simulink model "oc4_VarMass"  (R2026a)
settings: Solver=ode4  StartTime=0  StopTime=400  FixedStep=0.1  MaxStep=0.1  EnableMultiTasking=on
values from neighbouring files (symbols this model uses):
  simu = simulationClass()    [wecSimInputFile.m]
  waves = waveClass('regular')    [wecSimInputFile.m]
undefined symbols (not defined in the file or in its folder): body, constraint, X, Y, Z
libraries: nesl_utility x22, sm_lib x12, WECSim_Lib_Body_Elements x4, vrlib x1, matrix_library x1, WECSim_Lib_Constraints x1, WECSim_Lib_Frames x1
(part 1 of 3)
settings Model: Creator=mlawson  LastModifiedBy=jniffene
settings SolverCC: ZeroCrossControl=DisableAll  AlgebraicLoopSolver=LineSearch
settings OptimizationCC: SimCompilerOptimization=on
settings HardwareCC: ProdHWDeviceType=32-bit Generic
settings SimscapeCC: SimscapeNormalizeSystem=off  SimscapeNominalValues="[{\"value\":\"1\",\"unit\":\"A\"},{\"value\":\"1\",\"unit\":\"bar\"},{\"value\":\"1\",\"unit\":\"cm^2\"},{\"value\":\"1\",\"unit\":\"cm^3/s\"},{\"value\":\"1\",\"unit\":\"kJ/kg\"},{\"value\":\"1\",\"unit\":\"kW\"},{\"value\":\"1\",\"unit\":\"l\"},{\"value\":\"1\",\"unit\":\"N\"},{\"value\":\"1\",\"unit\":\"N*m\"},{\"value\":\"1\",\"unit\":\"V\"}]"  SimscapeLogType=none  SimscapeLogDataHistory=5000.0
settings ConfigurationSet: Description=SimMechanics 2G
settings ExplorerConfigSet: InternalSimMechanicsExplorerSettings="<ExplorerConfiguration><canonicalview>default</canonicalview><TilePanel><TileInfo><Tiles Columns=\"1\" Count=\"1\" Rows=\"1\"><Column Left=\"2\" Weight=\"1\"/><Column Left=\"1335\"/><Row Top=\"2\" Weight=\"1\"/><Row Top=\"911\"/><Tile Height=\"1\" Width=\"1\" X=\"0\" Y=\"0\"/></Tiles></TileInfo><SceneInfo><SceneViewer><BGColor><R>0.60000002384185791</R><G>0.60000002384185791</G><B>0.60000002384185791</B></BGColor><Camera><Position><X>365.37645888990272</X><Y>-369.82486814446582</Y><Z>359.64809521743916</Z></Position><Center><X>-6.7351450971904585</X><Y>2.2867358426280204</Y><Z>-12.463508769654169</Z></Center><Up><X>-0.40824829046386307</X><Y>0.40824829046386307</Y><Z>0.81649658092772615</Z></Up><Left>-57.820127362122818</Left><Right>57.820127362122818</Right><Bottom>-38.308817187253304</Bottom><Top>38.308817187253304</Top></Camera></SceneViewer></SceneInfo></TilePanel></ExplorerConfiguration>"

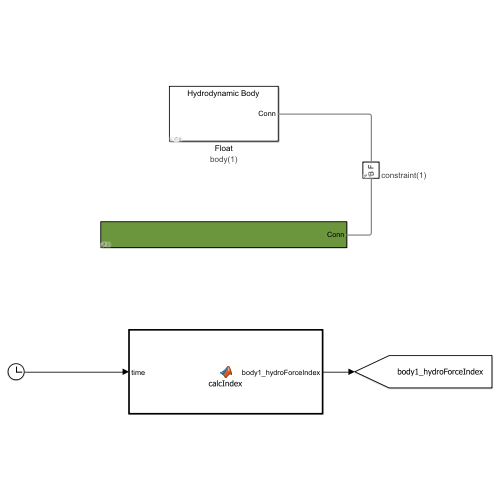
[thumbnail: Simulink's stored preview of the top-level diagram]
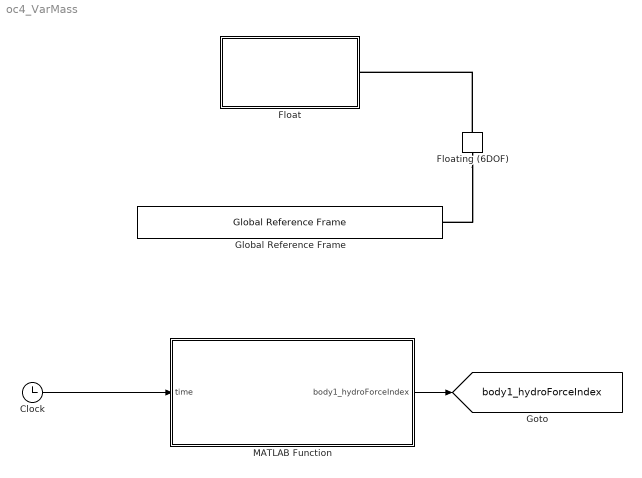
== system oc4_VarMass ==
  Clock : Clock
  Float : Subsystem  AncestorBlock=WECSim_Lib_Body_Elements/Rigid Body  Variant=on  EmptyChoice=on  mask(Rigid Body){body=body(1)}
      mask prompts: body "Body Number:"
      mask help:
      | A rigid body has no generalized body modes. It can be a standard hydrodynamic body, a drag body, or a non-hydrodynamic body.
      |
      | The variable name input below must be 'body(i)' where i=1,2,...
      | body(i) must be defined in the input file with the fields appropriate to each variant.
      mask init:
      | if exist('body','var')
      |     %%
      |     % Hydro Body
      |     h = [gcb '/Hydrodynamic Body'];
      |     responseName = ['sv_b' num2str(body.number) '_hydroBody'];
      |     set_param(h,'VariantControl',responseName);
      |     %%
      |     % Hydro Body Morison Element: Off
      |     h = [gcb '/Hydrodynamic Body/Morison Element and Viscous Damping Force Calculation/Morison Element Variant Subsystem/Morison Element Off'];
      |     responseName = ['sv_b' num2str(body.number) '_MEOff'];
      |     set_param(h,'VariantControl',responseName);
      |     %%
      |     % Hydro Body Morison Element: On
      |     h = [gcb '/Hydrodynamic Body/Morison Element and Viscous Damping Force Calculation/Morison Element Variant Subsystem/Morison Element On'];
      |     responseName = ['sv_b' num2str(body.number) '_MEOn'];
      |     set_param(h,'VariantControl',responseName);
      |     %%
      |     % Hydro Body Nonlinear Froude Krylov Force: Off
      |     h = [gcb '/Hydrodynamic Body/Wave Diffraction and Excitation Force Calculation/Nonlinear FK Force Variant Subsystem/No Nonlinear FroudeKrylov Force'];
      |     responseName = ['sv_b' num2str(body.number) '_linearHydro'];
      |     set_param(h,'VariantControl',responseName);
      |     %%
      |     % Hydro Body Nonlinear Froude Krylov Force: On
      |     h = [gcb '/Hydrodynamic Body/Wave Diffraction and Excitation Force Calculation/Nonlinear FK Force Variant Subsystem/With Nonlinear FroudeKrylov Force'];
      |     responseName = ['sv_b' num2str(body.number) '_nonlinearHydro'];
      |     set_param(h,'VariantControl',responseName);
      |     %%
      |     % Hydro Body Nonlinear Restoring: Off
      |     h = [gcb '/Hydrodynamic Body/Hydrostatic Restoring Force Calculation/Linear and Nonlinear Restoring Force Variant Subsystem/Linear Hydrostatic Restoring Force'];
      |     responseName = ['sv_b' num2str(body.number) '_linearHydro'];
      |     set_param(h,'VariantControl',responseName);
      |     %%
      |     % Hydro Body Nonlinear Restoring: On
      |     h = [gcb '/Hydrodynamic Body/Hydrostatic Restoring Force Calculation/Linear and Nonlinear Restoring Force Variant Subsystem/Nonlinear Hydrostatic Restoring Force'];
      |     responseName = ['sv_b' num2str(body.number) '_nonlinearHydro'];
      |     set_param(h,'VariantControl',responseName);
      |     %%
      |     % Hydro Body Regular Excitation Passive Yaw: Off
      |     h = [gcb '/Hydrodynamic Body/Wave Diffraction and Excitation Force Calculation/Linear Wave Excitation Force Variant Subsystem/Regular Wave ' newline 'Excitation Force'];
      |     responseName = ['sv_regularWaves_b' num2str(body.number)];
      |     set_param(h,'VariantControl',responseName);
      |     %%
      |     % Hydro Body Regular Excitation Passive Yaw: On
      |     h = [gcb '/Hydrodynamic Body/Wave Diffraction and Excitation Force Calculation/Linear Wave Excitation Force Variant Subsystem/Regular Wave ' newline 'NonLinear Yaw'];
      |     responseName = ['sv_regularWavesYaw_b' num2str(body.number)];
      |     set_param(h,'VariantControl',responseName);
      |     %%    
      |     % Hydro Body Irregular Excitation Passive Yaw: Off
      |     h = [gcb '/Hydrodynamic Body/Wave Diffraction and Excitation Force Calculation/Linear Wave Excitation Force Variant Subsystem/Irregular Wave ' newline 'Excitation Force'];
      |     responseName = ['sv_irregularWaves_b' num2str(body.number)];
      |     set_param(h,'VariantControl',responseName);
      |     %%
      |     % Hydro Body Irregular Excitation Passive Yaw: On
      |     h = [gcb '/Hydrodynamic Body/Wave Diffraction and Excitation Force Calculation/Linear Wave Excitation Force Variant Subsystem/Irregular Wave ' newline 'NonLinearYaw'];
      |     responseName = ['sv_irregularWavesYaw_b' num2str(body.number)];
      |     set_param(h,'VariantControl',responseName);
      |     %%
      |     % Hydro Body Nonlinear Froude Krylov or Restoring: Instantaneous Free Surface
      |     h = [gcb '/Hydrodynamic Body/Nonlinear Wave Elevation/Linear or Instantaneous Free Surface/Instantaneous Water Free Surface'];
      |     responseName = ['sv_b' num2str(body.number) '_instFS'];
      |     set_param(h,'VariantControl',responseName);
      |     %%
      |     % Hydro Body Nonlinear Froude Krylov or Restoring: Mean Free Surface
      |     h = [gcb '/Hydrodynamic Body/Nonlinear Wave Elevation/Linear or Instantaneous Free Surface/Mean Water Free Surface'];
      |     responseName = ['sv_b' num2str(body.number) '_meanFS'];
      |     set_param(h,'VariantControl',responseName);
      |     %% Variable hydro on/off
      |     % Variable hydro control - variable hydro off
      |     h = [gcb '/Hydrodynamic Body/Variable Hydrodynamics Control/Variable Hydrodynamics Subsystem/noVariableHydro'];
      |     responseName = ['sv_b' num2str(body.number) '_noVariableHydro'];
      |     set_param(h,'VariantControl',responseName);
      |     % Variable hydro control - variable hydro on
      |     h = [gcb '/Hydrodynamic Body/Variable Hydrodynamics Control/Variable Hydrodynamics Subsystem/variableHydro'];
      |     responseName = ['sv_b' num2str(body.number) '_variableHydro'];
      |     set_param(h,'VariantControl',responseName);
      |     % CIC - variable hydro off
      |     h = [gcb '/Hydrodynamic Body/Wave Radiation Forces Calculation/SS CI and Constant-Damping-CoeVariant Subsystem/Convolution Integral Calculation/Convolution Variant Subsystem/Convolution Integral Calculation'];
      |     responseName = ['sv_b' num2str(body.number) '_noVariableHydro'];
      |     set_param(h,'VariantControl',responseName);
      |     % CIC - variable hydro on
      |     h = [gcb '/Hydrodynamic Body/Wave Radiation Forces Calculation/SS CI and Constant-Damping-CoeVariant Subsystem/Convolution Integral Calculation/Convolution Variant Subsystem/Convolution Integral Surface Calculation'];
      |     responseName = ['sv_b' num2str(body.number) '_variableHydro'];
      |     set_param(h,'VariantControl',responseName);
      |     %%
      |     % Drag Body
      |     h = [gcb '/Drag Body'];
      |     responseName = ['sv_b' num2str(body.number) '_dragBody'];
      |     set_param(h,'VariantControl',responseName);
      |     %%
      |     % Drag Body Morison Element: Off
      |     h = [gcb '/Drag Body/Morison Element and Viscous Damping Force Calculation/Morison Element Variant Subsystem/Morison Element Off'];
      |     responseName = ['sv_b' num2str(body.number) '_MEOff'];
      |     set_param(h,'VariantControl',responseName);
      |     %%
      |     % Drag Body Morison Element: On
      |     h = [gcb '/Drag Body/Morison Element and Viscous Damping Force Calculation/Morison Element Variant Subsystem/Morison Element On'];
      |     responseName = ['sv_b' num2str(body.number) '_MEOn'];
      |     set_param(h,'VariantControl',responseName);
      |     %% 
      |     % Hydro Body QTF: Off
      |     h = [gcb '/Hydrodynamic Body/Wave Diffraction and Excitation Force Calculation/Second Order Excitation Force Variant Subsystem/No Second Order Excitation Force'];
      |     responseName = ['sv_b' num2str(body.number) '_noSecondOrderExt'];
      |     set_param(h,'VariantControl',responseName);
      |     %%
      |     % Hydro Body QTF: On
      |     h = [gcb '/Hydrodynamic Body/Wave Diffraction and Excitation Force Calculation/Second Order Excitation Force Variant Subsystem/With Second Order Excitation Force'];
      |     responseName = ['sv_b' num2str(body.number) '_secondOrderExt'];
      |     set_param(h,'VariantControl',responseName);
      |     %%
      |     % Set zero active variant controls to prevent label issue
      |     set_param(gcb,'AllowZeroVariantControls','on');
      | end
      | clear bc h geomFile responseName
      settings: AttributesFormatString=%<body>
      mask Help:
      | A rigid body has no generalized body modes. It can be a standard hydrodynamic body, a drag body, or a non-hydrodynamic body.
      | 
      | The variable name input below must be 'body(i)' where i=1,2,...
      | body(i) must be defined in the input file with the fields appropriate to each variant.
  Floating (6DOF) : WECSim_Lib_Constraints/Floating (6DOF)  constraint=constraint(1)
      settings: AttributesFormatString=%<constraint>
  Global Reference Frame : WECSim_Lib_Frames/Global Reference Frame  waves=waves  simu=simu
  MATLAB Function : MATLAB Function  TreatAsAtomicUnit=on
  tag scope: body1_hydroForceIndex=global
  wires:
  MATLAB Function/1(body1_hydroForceIndex) -> [body1_hydroForceIndex]
  Clock/1 -> MATLAB Function/1(time)
  connections:
  Floating (6DOF)/LConn1 -- Global Reference Frame/RConn1
  Floating (6DOF)/RConn1 -- Float/RConn1

== system oc4_VarMass/Float ==
  note: 1) Add Subsystem or Model blocks as valid variant choices.
      | 2) You cannot connect blocks at this level. At simulation, connectivity is automatically
      | determined, based on the active variant and port name matching.
  Drag Body : Subsystem  VariantControl=sv_b1_dragBody  mask(Drag Body){body=body}
      mask prompts: body "Body Name:"
      mask help:
      | A drag body contains six degrees of freedom in x, y, z and Mx, My, Mz. It contains a buoyant force, linear damping force, and Morison Element and viscous forces. It is not influenced by wave excitation, radiation damping or radiation added mass.
      |
      | The variable name input below must be 'body(i)' where i=1,2,...
      | body(i) must be defined in the input file with the following fields:
      |
      |     .mass (required)
      |             Float or string.
      |             The translational interia or mass of the body in kg. If a string, the value must be 'equilibrium'. Default = [ ]
      |     .momOfIntertia (required)
      |             3x1 vector [Ixx Iyy Izz].
      |             Rotational intertia of the body in kg*m^2. Default = [ ]
      |     .filename (required)
      |             String.
      |             The file path specifying the .h5 file for the body.
      |     .name (optional)
      |             String.
      |             Specifies the body name. Default = [ ]
      |     .cg (optional)
      |             3x1 float vector [x y z]
      |     .cb (optional)
      |             3x1 float vector [x y z]
      |             Body center of buoyancy in m. Default = [ ].
      |     .dispVol (optional)
      |             Float.
      |             Displaced volume at the equilibrium position in m^3. Default = [ ]
      |     .geometryFile (optional)
      |             String
      |             Path to the geometry file of the body (.stl). Required for nonlinear hydrodynamics or visualization. Default = [ ]
      mask init:
      | if exist('body','var')
      |     % geometry file name
      |     h=[gcb '/Structure/Body Properties'];
      |     geomFile=body.geometryFile;
      |     set_param(h,'ExtGeomFileName',geomFile);
      |     geomType='STL';
      |     % split version e.g. '9.10.0.16028 (R2021a)' into 9, 10, 0, NaN.
      |     % cannot compare str2double('9.10') because it becomes '9.1' 
      |     ver=split(version,'.');
      |     ver=str2double(ver(1:3));
      |     if ver(1) < 9 || (ver(1) == 9 && ver(2) < 6)
      |        set_param(h,'ExtGeomFileType',geomType);
      |     end
      |     % toWorkSpace: outputs
      |     h=[gcb '/To Workspace'];
      |     responseName=['body' num2str(body.number) '_out'];
      |     set_param(h,'VariableName',responseName);
      |     % position GoTo 
      |     h=[gcb '/Goto'];
      |     responseName=['disp' num2str(body.number)];
      |     set_param(h,'GotoTag',responseName);
      |     % position From
      |     h=[gcb '/From'];
      |     responseName=['disp' num2str(body.number)];
      |     set_param(h,'GotoTag',responseName);
      |     % velocity GoTo 
      |     h=[gcb '/Goto1'];
      |     responseName=['vel' num2str(body.number)];
      |     set_param(h,'GotoTag',responseName);
      |     % velocity From 
      |     h=[gcb '/From1'];
      |     responseName=['vel' num2str(body.number)];
      |     set_param(h,'GotoTag',responseName);
      |     % acceleration GoTo 
      |     h=[gcb '/Goto2'];
      |     responseName=['acc' num2str(body.number)];
      |     set_param(h,'GotoTag',responseName);
      |     % acceleration From 
      |     h=[gcb '/From2'];
      |     responseName=['acc' num2str(body.number)];
      |     set_param(h,'GotoTag',responseName);
      | end
  Hydrodynamic Body : Subsystem  VariantControl=sv_b1_hydroBody  mask(Hydrodynamic Body){body=body}
      mask prompts: body "Body Name:"
      mask help:
      | A Hydrodynamic Body contains six degrees of freedom in x, y, z and Mx, My, Mz. All wave forces interact with a hydrodynamic body.
      |
      | The variable name input below must be 'body(i)' where i=1,2,...
      | body(i) must be defined in the input file with the following fields:
      |
      |     .filename (required)
      |             String.
      |             The file path specifying the .h5 file for the body.
      |     .mass (required)
      |             Float or string.
      |             The translational interia or mass of the body in kg. If a string, the value must be 'equilibrium'. Default = [ ]
      |     .momOfIntertia (required)
      |             3x1 vector [Ixx Iyy Izz].
      |             Rotational intertia of the body in kg*m^2. Default = [ ]
      |     .geometryFile (optional)
      |             String
      |             Path to the geometry file of the body (.stl). Required for nonlinear hydrodynamics or visualization. Default = [ ]
      mask init:
      | if exist('body','var') && ~isempty(body)
      |     % geometry file name
      |     h=[gcb '/Structure/Body Properties'];
      |     geomFile=body.geometryFile;
      |     set_param(h,'ExtGeomFileName',geomFile);
      |     geomType='STL';
      |     % split version e.g. '9.10.0.16028 (R2021a)' into 9, 10, 0, NaN.
      |     % cannot compare str2double('9.10') because it becomes '9.1' 
      |     ver=split(version,'.');
      |     ver=str2double(ver(1:3));
      |     if ver(1) < 9 || (ver(1) == 9 && ver(2) < 6)
      |        set_param(h,'ExtGeomFileType',geomType);
      |     end
      |     % toWorkSpace: outputs
      |     h=[gcb '/To Workspace'];
      |     responseName=['body' num2str(body.number) '_out'];
      |     set_param(h,'VariableName',responseName);
      |     % toWorkSpace: hydrostatic pressures
      |     h=[gcb '/Hydrostatic Restoring Force Calculation/Linear and Nonlinear Restoring Force Variant Subsystem/Nonlinear Hydrostatic Restoring Force/To Workspace1'];
      |     responseName=['body' num2str(body.number) '_hspressure_out'];
      |     set_param(h,'VariableName',responseName); 
      |     % toWorkSpace: wave pressures (non-linear Freude-Krylov)
      |     h=[gcb '/Wave Diffraction and Excitation Force Calculation/Nonlinear FK Force Variant Subsystem/With Nonlinear FroudeKrylov Force/To Workspace'];
      |     responseName=['body' num2str(body.number) '_wavenonlinearpressure_out'];
      |     set_param(h,'VariableName',responseName);
      |     % toWorkSpace: wave pressures (linear Freude-Krylov)
      |     h=[gcb '/Wave Diffraction and Excitation Force Calculation/Nonlinear FK Force Variant Subsystem/With Nonlinear FroudeKrylov Force/To Workspace1'];
      |     responseName=['body' num2str(body.number) '_wavelinearpressure_out'];
      |     set_param(h,'VariableName',responseName);
      | 
      |     % position GoTo 
      |     h=[gcb '/Goto'];
      |     responseName=['disp' num2str(body.number)];
      |     set_param(h,'GotoTag',responseName);
      |     % position From
      |     h=[gcb '/From'];
      |     responseName=['disp' num2str(body.number)];
      |     set_param(h,'GotoTag',responseName);
      | 
      |     % velocity GoTo 
      |     h=[gcb '/Goto1'];
      |     responseName=['vel' num2str(body.number)];
      |     set_param(h,'GotoTag',responseName);
      |     % velocity From 
      |     h=[gcb '/From1'];
      |     responseName=['vel' num2str(body.number)];
      |     set_param(h,'GotoTag',responseName);
      | 
      |     % acceleration GoTo
      |     h=[gcb '/Goto2'];
      |     responseName=['acc' num2str(body.number)];
      |     set_param(h,'GotoTag',responseName);
      |     % acceleration From 
      |     h=[gcb '/From2'];
      |     responseName=['acc' num2str(body.number)];
      |     set_param(h,'GotoTag',responseName);
      | 
      |     % excitation force GoTo
      |     h = [gcb '/Goto3'];
      |     responseName = ['b' num2str(body.number) '_f_excitation'];
      |     set_param(h, 'GotoTag', responseName);
      |     % total force GoTo
      |     h = [gcb '/Goto4'];
      |     responseName = ['b' num2str(body.number) '_f_total'];
      |     set_param(h, 'GotoTag', responseName);
      |     
      |     %% Variable Hydro:
      |     % Variant subsystem
      |     h = [gcb '/Variable Hydrodynamics Control/Variable Hydrodynamics Subsystem'];
      |     responseName = ['sv_b' num2str(body.number) '_variableHydro'];
      |     set_param(h,'VariantControl',responseName);
      |     % body_hydroForceIndex To Workspace tags
      |     h=[gcb '/Variable Hydrodynamics Control/Variable Hydrodynamics Subsystem/variableHydro/To Workspace'];
      |     responseName=['body' num2str(body.number) '_hydroForceIndex'];
      |     set_param(h,'VariableName',responseName); 
      |     % body_hydroForceIndex From tags
      |     h=[gcb '/Variable Hydrodynamics Control/Variable Hydrodynamics Subsystem/variableHydro/From'];
      |     responseName=['body' num2str(body.number) '_hydroForceIndex'];
      |     set_param(h,'GotoTag',responseName);
      |     h=[gcb '/Wave Radiation Forces Calculation/SS CI and Constant-Damping-CoeVariant Subsystem/Convolution Integral Calculation/Convolution Variant Subsystem/Convolution Integral Surface Calculation/From'];
      |     responseName=['body' num2str(body.number) '_hydroForceIndex'];
      |     set_param(h,'GotoTag',responseName);
      |     % body_hydroForce GoTo
      |     h=[gcb '/Variable Hydrodynamics Control/Goto'];
      |     responseName=['body' num2str(body.number) '_hydroForce'];
      |     set_param(h,'GotoTag',responseName);
      |     % body_hydroForce From tags
      |     h=[gcb '/Wave Diffraction and Excitation Force Calculation/From'];
      |     responseName=['body' num2str(body.number) '_hydroForce'];
      |     set_param(h,'GotoTag',responseName);
      |     h=[gcb '/Wave Radiation Forces Calculation/From'];
      |     responseName=['body' num2str(body.number) '_hydroForce'];
      |     set_param(h,'GotoTag',responseName);
      |     h=[gcb '/Wave Radiation Forces Calculation/SS CI and Constant-Damping-CoeVariant Subsystem/Constant Coefficients/From'];
      |     responseName=['body' num2str(body.number) '_hydroForce'];
      |     set_param(h,'GotoTag',responseName);
      |     h=[gcb '/Wave Radiation Forces Calculation/SS CI and Constant-Damping-CoeVariant Subsystem/Convolution Integral Calculation/Convolution Variant Subsystem/Convolution Integral Calculation/From'];
      |     responseName=['body' num2str(body.number) '_hydroForce'];
      |     set_param(h,'GotoTag',responseName);
      |     h=[gcb '/Hydrostatic Restoring Force Calculation/Linear and Nonlinear Restoring Force Variant Subsystem/Linear Hydrostatic Restoring Force/From'];
      |     responseName=['body' num2str(body.number) '_hydroForce'];
      |     set_param(h,'GotoTag',responseName);
      |     h=[gcb '/Hydrostatic Restoring Force Calculation/Linear and Nonlinear Restoring Force Variant Subsystem/Nonlinear Hydrostatic Restoring Force/From'];
      |     responseName=['body' num2str(body.number) '_hydroForce'];
      |     set_param(h,'GotoTag',responseName);
      |     h=[gcb '/Hydrostatic Restoring Force Calculation/From'];
      |     responseName=['body' num2str(body.number) '_hydroForce'];
      |     set_param(h,'GotoTag',responseName);
      |     h=[gcb '/From3'];
      |     responseName=['body' num2str(body.number) '_hydroForce'];
      |     set_param(h,'GotoTag',responseName);
      |     % Update body.hydroForce constant data type
      |     h=[gcb '/Variable Hydrodynamics Control/Constant'];
      |     busName=['Bus: bus_body' num2str(body.number) '_hydroForce'];
      |     set_param(h,'OutDataTypeStr',busName);
      | end
  Conn : PMIOPort  Side=Right

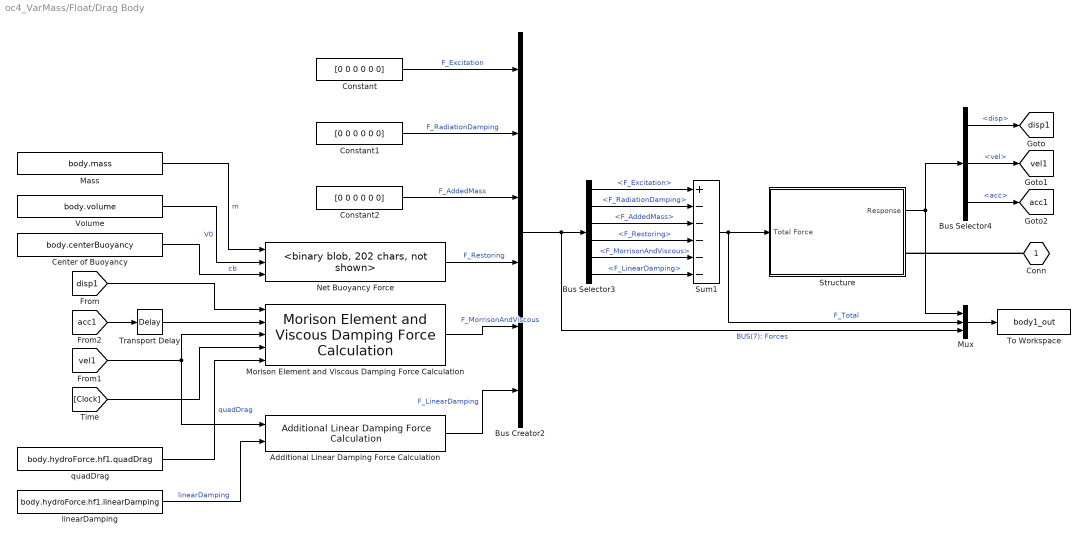
== system oc4_VarMass/Float/Drag Body ==
  Additional Linear Damping Force Calculation : WECSim_Lib_Body_Elements/Rigid Body/Hydrodynamic Body/Additional Linear Damping Force Calculation  SystemSampleTime=-1  VariantActivationTime=update diagram  Latency=0  AutoFrameSizeCalculation=off
  Bus Creator2 : BusCreator  Inputs=6
  Bus Selector3 : BusSelector  OutputSignals=F_Excitation,F_RadiationDamping,F_AddedMass,F_Restoring,F_MorrisonAndViscous,F_LinearDamping
  Bus Selector4 : BusSelector  OutputSignals=disp,vel,acc
  Center of Buoyancy : Constant  Value=body.centerBuoyancy
  Constant : Constant  Value=[0 0 0 0 0 0]
  Constant1 : Constant  Value=[0 0 0 0 0 0]
  Constant2 : Constant  Value=[0 0 0 0 0 0]
  Mass : Constant  Value=body.mass
  Morison Element and Viscous Damping Force Calculation : WECSim_Lib_Body_Elements/Rigid Body/Hydrodynamic Body/Morison Element and Viscous Damping Force Calculation  SystemSampleTime=-1  VariantActivationTime=update diagram  EmptyChoice=off  PassThrough=off  PassThroughVariantControl=(default)  EmptyChoiceVariantControl=(default)  AllowFlexibleInterface=on  Latency=0  AutoFrameSizeCalculation=off
  Mux : Mux  Inputs=3
  Net Buoyancy Force : WECSim_Lib_Body_Elements/Rigid Body/Hydrodynamic Body/Hydrostatic Restoring Force Calculation/Linear and Nonlinear Restoring Force Variant Subsystem/Linear Hydrostatic Restoring Force/Net Buoyancy Force  SystemSampleTime=-1  VariantActivationTime=update diagram  Latency=0  AutoFrameSizeCalculation=off
  Structure : Subsystem
  Sum1 : Sum  Inputs=+-----
  To Workspace : ToWorkspace  VariableName=body1_out  SaveFormat=Structure With Time  SampleTime=simu.dtOut
  Transport Delay : TransportDelay  DelayTime=10e-8
  Volume : Constant  Value=body.volume
  linearDamping : Constant  Value=body.hydroForce.hf1.linearDamping
  quadDrag : Constant  Value=body.hydroForce.hf1.quadDrag
  Conn : PMIOPort  Side=Right
  tag scope: acc1=global, disp1=global, vel1=global
  wires:
  linearDamping/1 -> Additional Linear Damping Force Calculation/2  "linearDamping"
  quadDrag/1 -> Morison Element and Viscous Damping Force Calculation/5  "quadDrag"
  Mass/1 -> Net Buoyancy Force/1  "m"
  Volume/1 -> Net Buoyancy Force/2  "V0"
  Center of Buoyancy/1 -> Net Buoyancy Force/3  "cb"
  [disp1] -> Morison Element and Viscous Damping Force Calculation/1
  [Clock] -> Morison Element and Viscous Damping Force Calculation/4
  [vel1] -> Additional Linear Damping Force Calculation/1, Morison Element and Viscous Damping Force Calculation/3
  Transport Delay/1 -> Morison Element and Viscous Damping Force Calculation/2
  Bus Selector4/3 -> [acc1]  "<acc>"
  Structure/1(Response) -> Bus Selector4/1, Mux/1
  Bus Selector4/2 -> [vel1]  "<vel>"
  Bus Selector4/1 -> [disp1]  "<disp>"
  Bus Selector3/6 -> Sum1/6  "<F_LinearDamping>"
  Bus Selector3/2 -> Sum1/2  "<F_RadiationDamping>"
  Constant2/1 -> Bus Creator2/3  "F_AddedMass"
  Sum1/1 -> Structure/1(Total Force), Mux/2  "F_Total"
  Bus Creator2/1 -> Bus Selector3/1, Mux/3  "BUS(7): Forces"
  Bus Selector3/3 -> Sum1/3  "<F_AddedMass>"
  Bus Selector3/4 -> Sum1/4  "<F_Restoring>"
  Constant/1 -> Bus Creator2/1  "F_Excitation"
  Morison Element and Viscous Damping Force Calculation/1 -> Bus Creator2/5  "F_MorrisonAndViscous"
  Additional Linear Damping Force Calculation/1 -> Bus Creator2/6  "F_LinearDamping"
  Net Buoyancy Force/1 -> Bus Creator2/4  "F_Restoring"
  Mux/1 -> To Workspace/1
  Constant1/1 -> Bus Creator2/2  "F_RadiationDamping"
  Bus Selector3/5 -> Sum1/5  "<F_MorrisonAndViscous>"
  Bus Selector3/1 -> Sum1/1  "<F_Excitation>"
  [acc1] -> Transport Delay/1
  connections:
  Conn/RConn1 -- Structure/RConn1

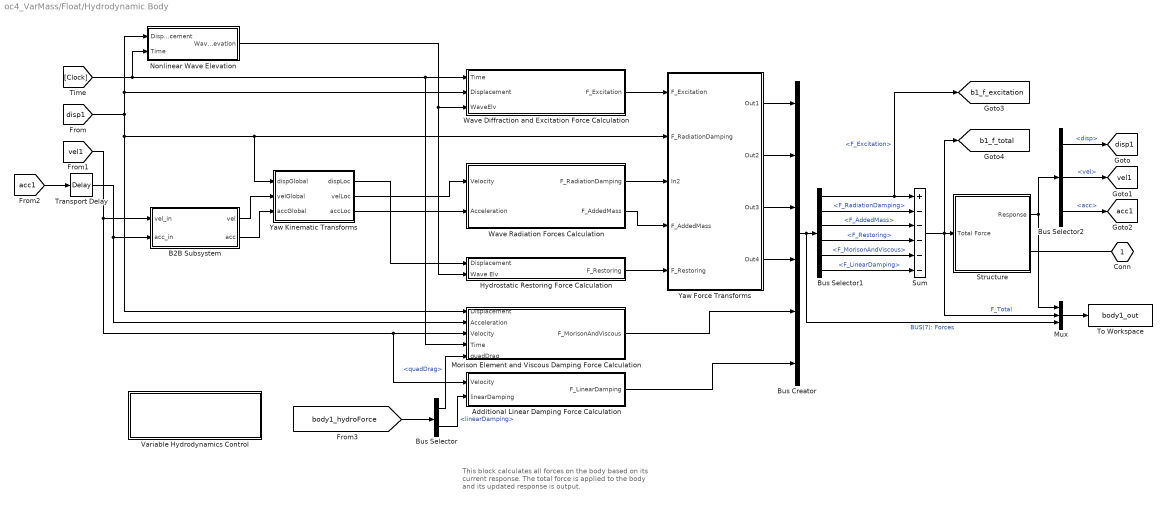
== system oc4_VarMass/Float/Hydrodynamic Body ==
  note: This block calculates all forces on the body based on its current response. The total force is applied to the body and its updated response is output.
  Additional Linear Damping Force Calculation : Subsystem
  B2B Subsystem : Subsystem  Variant=on
  Bus Creator : BusCreator  Inputs=6
  Bus Selector : BusSelector  OutputSignals=quadDrag,linearDamping
  Bus Selector1 : BusSelector  OutputSignals=F_Excitation,F_RadiationDamping,F_AddedMass,F_Restoring,F_MorisonAndViscous,F_LinearDamping
  Bus Selector2 : BusSelector  OutputSignals=disp,vel,acc
  Hydrostatic Restoring Force Calculation : Subsystem
  Morison Element and Viscous Damping Force Calculation : Subsystem
  Mux : Mux  Inputs=3
  Nonlinear Wave Elevation : Subsystem  TreatAsAtomicUnit=on  SystemSampleTime=simu.nonlinearDt
  Structure : Subsystem
  Sum : Sum  Inputs=+-----
  To Workspace : ToWorkspace  VariableName=body1_out  SaveFormat=Structure With Time  SampleTime=simu.dtOut
  Transport Delay : TransportDelay  DelayTime=10e-8
  Variable Hydrodynamics Control : Subsystem  mask{body=body}
      mask prompts: body "Body Name:"
  Wave Diffraction and Excitation Force Calculation : Subsystem  mask{waveGroup=waves}
      mask prompts: waveGroup "Waves Object"
      mask init:
      | cb = gcb;
      | nWaves = size(waveGroup,2);
      | for iWG = 2:nWaves
      |     try 
      |         find_system([cb,'/Linear Wave Excitation Force Variant Subsystem',num2str(iWG)],'Type','Block');
      |     catch
      |         % Duplicate the linear excitation force block for multiple waves
      |         add_block([cb,'/Linear Wave Excitation Force Variant Subsystem'],[cb,'/Linear Wave Excitation Force Variant Subsystem',num2str(iWG)],'MakeNameUnique','off',...
      |                    'Position',[400,200*iWG,580,40+200*iWG],'BackgroundColor','white');
      |         set_param([cb,'/Linear Wave Excitation Force Variant Subsystem',num2str(iWG)],...
      |                'Nwave',sprintf('waves(%d)',iWG) );
      | 
      |         % Connect lines to the new block
      |         add_line(cb,...
      |            ['FexcInputs/1'],...
      |            ['Linear Wave Excitation Force Variant Subsystem',num2str(iWG),'/1'],...
      |            'autorouting','on');
      |         add_line(cb,...
      |            ['FexcInputs/2'],...
      |            ['Linear Wave Excitation Force Variant Subsystem',num2str(iWG),'/2'],...
      |            'autorouting','on');
      |         add_line(cb,...
      |            ['FexcInputs/4'],...
      |            ['Linear Wave Excitation Force Variant Subsystem',num2str(iWG),'/3'],...
      |            'autorouting','on');
      |         signlist = get_param([cb,'/Add'],'Inputs');   
      |         set_param([cb,'/Add'],'Inputs',[signlist,'+']);
      |         add_line(cb,...
      |         ['Linear Wave Excitation Force Variant Subsystem',num2str(iWG),'/1'],...
      |         sprintf('Add/%d',length(signlist)+1),...
      |         'autorouting','on');
      |     end
      | end
  Wave Radiation Forces Calculation : Subsystem
  Yaw Force Transforms : Subsystem
  Yaw Kinematic Transforms : Subsystem  Variant=on
  Conn : PMIOPort  Side=Right
  tag scope: acc1=global, b1_f_excitation=global, b1_f_total=global, disp1=global, vel1=global
  wires:
  Bus Selector/2 -> Additional Linear Damping Force Calculation/2(linearDamping)  "<linearDamping>"
  Bus Selector/1 -> Morison Element and Viscous Damping Force Calculation/5(quadDrag)  "<quadDrag>"
  [body1_hydroForce] -> Bus Selector/1
  Yaw Force Transforms/3(Out3) -> Bus Creator/3
  Yaw Force Transforms/4(Out4) -> Bus Creator/4
  Yaw Force Transforms/2(Out2) -> Bus Creator/2
  Yaw Force Transforms/1(Out1) -> Bus Creator/1
  Wave Radiation Forces Calculation/1(F_RadiationDamping) -> Yaw Force Transforms/3(In2)
  Mux/1 -> To Workspace/1
  [vel1] -> Morison Element and Viscous Damping Force Calculation/3(Velocity), Additional Linear Damping Force Calculation/1(Velocity), B2B Subsystem/1(vel_in)
  Nonlinear Wave Elevation/1(Wave Elevation) -> Hydrostatic Restoring Force Calculation/2(Wave Elv), Wave Diffraction and Excitation Force Calculation/3(WaveElv)
  Yaw Kinematic Transforms/2(velLoc) -> Wave Radiation Forces Calculation/1(Velocity)
  Yaw Kinematic Transforms/1(dispLoc) -> Hydrostatic Restoring Force Calculation/1(Displacement)
  B2B Subsystem/1(vel) -> Yaw Kinematic Transforms/2(velGlobal)
  Bus Selector2/3 -> [acc1]  "<acc>"
  Transport Delay/1 -> Morison Element and Viscous Damping Force Calculation/2(Acceleration), B2B Subsystem/2(acc_in)
  Additional Linear Damping Force Calculation/1(F_LinearDamping) -> Bus Creator/6
  [Clock] -> Morison Element and Viscous Damping Force Calculation/4(Time), Wave Diffraction and Excitation Force Calculation/1(Time), Nonlinear Wave Elevation/2(Time)
  Yaw Kinematic Transforms/3(accLoc) -> Wave Radiation Forces Calculation/2(Acceleration)
  [acc1] -> Transport Delay/1
  Bus Selector2/1 -> [disp1]  "<disp>"
  Sum/1 -> Structure/1(Total Force), Mux/2, [b1_f_total]  "F_Total"
  Bus Selector2/2 -> [vel1]  "<vel>"
  B2B Subsystem/2(acc) -> Yaw Kinematic Transforms/3(accGlobal)
  Bus Creator/1 -> Bus Selector1/1, Mux/3  "BUS(7): Forces"
  Structure/1(Response) -> Bus Selector2/1, Mux/1
  Morison Element and Viscous Damping Force Calculation/1(F_MorisonAndViscous) -> Bus Creator/5
  Wave Radiation Forces Calculation/2(F_AddedMass) -> Yaw Force Transforms/4(F_AddedMass)
  Wave Diffraction and Excitation Force Calculation/1(F_Excitation) -> Yaw Force Transforms/1(F_Excitation)
  [disp1] -> Morison Element and Viscous Damping Force Calculation/1(Displacement), Yaw Force Transforms/2(F_RadiationDamping), Yaw Kinematic Transforms/1(dispGlobal), Wave Diffraction and Excitation Force Calculation/2(Displacement), Nonlinear Wave Elevation/1(Displacement)
  Hydrostatic Restoring Force Calculation/1(F_Restoring) -> Yaw Force Transforms/5(F_Restoring)
  Bus Selector1/1 -> Sum/1, [b1_f_excitation]  "<F_Excitation>"
  Bus Selector1/2 -> Sum/2  "<F_RadiationDamping>"
  Bus Selector1/3 -> Sum/3  "<F_AddedMass>"
  Bus Selector1/4 -> Sum/4  "<F_Restoring>"
  Bus Selector1/5 -> Sum/5  "<F_MorisonAndViscous>"
  Bus Selector1/6 -> Sum/6  "<F_LinearDamping>"
  connections:
  Conn/RConn1 -- Structure/RConn1

== system oc4_VarMass/Float/Drag Body/Structure ==
  note: Apply the total force to the body and calculate its response relative to the global reference frame.
      |
      | Output force to apply to another body.
  Total Force : Inport
  Body Properties : sm_lib/Body Elements/File Solid  ExtGeomFileName=../BEM/OC4_Semisub.stl  UnitType=Custom  ExtGeomFileUnits=m  StepReaderType=HEX  ExportConvexHullGeometry=off  InertiaType=Custom  BasedOnType=Density  Density=1000  DensityUnits=kg/(m^3)  Mass=body.mass  MassUnits=kg  CenterOfMass=[0 0 0]  CenterOfMassUnits=m  MomentsOfInertia=body.inertia  MomentsOfInertiaUnits=kg*m^2  ProductsOfInertia=body.inertiaProducts  ProductsOfInertiaUnits=kg*m^2  GraphicType=FromGeometry  MarkerShape=Sphere  MarkerSize=10  GraphicVisPropType=SimpleVisualProperties  GraphicDiffuseColor=body.viz.color  GraphicOpacity=body.viz.opacity  GraphicSpecularColor=[0.5 0.5 0.5 1.0]  GraphicAmbientColor=[0.15 0.15 0.15 1.0]  GraphicEmissiveColor=[0.0 0.0 0.0 1.0]  GraphicShininess=75  DoExposeReferenceFrame=on  SerializedFrames=<Frames/>
  External Force and Torque : sm_lib/Forces and Torques/External Force and Torque  ForceResolutionFrame=World  EnableForceX=off  EnableForceY=off  EnableForceZ=off  EnableForce=on  TorqueResolutionFrame=World  EnableTorqueX=off  EnableTorqueY=off  EnableTorqueZ=off  EnableTorque=on
  Motion Sensor : WECSim_Lib_Body_Elements/Rigid Body/Hydrodynamic Body/Structure/Motion Sensor  SystemSampleTime=-1  VariantActivationTime=update diagram  AllowFlexibleInterface=on  Latency=0  AutoFrameSizeCalculation=off
  Rigid Transform (Setup CG) : sm_lib/Frames and Transforms/Rigid Transform  TranslationMethod=Cartesian  TranslationStandardOffset=0  TranslationStandardOffsetUnits=m  TranslationStandardAxis=+Z  TranslationCartesianOffset=body.centerGravity  TranslationCartesianOffsetUnits=m  TranslationROffset=0  TranslationROffsetUnits=m  TranslationZOffset=0  TranslationZOffsetUnits=m  TranslationThetaOffset=0  TranslationThetaOffsetUnits=deg  RotationMethod=None  RotationAngleUnits=rad  RotationStandardAxis=+Y  RotationAngle=0.05  RotationArbitraryAxis=[0.57735026918962584 0.57735026918962584 0.57735026918962584]  FollAlignAxisA=+X  BaseAlignAxisA=+Y  FollAlignAxisB=+Y  BaseAlignAxisB=+Z  RotationSequenceAxes=FollowerAxes  RotationSequence=XYX  RotationSequenceAngles=[0 0 0]  RotationSequenceAnglesUnits=deg  RotationMatrix=[1 0 0; 0 1 0; 0 0 1]  Quaternion=[1 0 0 0]
  Rigid Transform (Setup Initial Disp) : sm_lib/Frames and Transforms/Rigid Transform  TranslationMethod=Cartesian  TranslationStandardOffset=0  TranslationStandardOffsetUnits=m  TranslationStandardAxis=+Z  TranslationCartesianOffset=body.initial.displacement  TranslationCartesianOffsetUnits=m  TranslationROffset=0  TranslationROffsetUnits=m  TranslationZOffset=0  TranslationZOffsetUnits=m  TranslationThetaOffset=0  TranslationThetaOffsetUnits=deg  RotationMethod=ArbitraryAxis  RotationAngleUnits=rad  RotationStandardAxis=+Y  RotationAngle=body.initial.angle  RotationArbitraryAxis=body.initial.axis  FollAlignAxisA=+X  BaseAlignAxisA=+Y  FollAlignAxisB=+Y  BaseAlignAxisB=+Z  RotationSequenceAxes=FollowerAxes  RotationSequence=XYX  RotationSequenceAngles=[0 0 0]  RotationSequenceAnglesUnits=deg  RotationMatrix=[1 0 0; 0 1 0; 0 0 1]  Quaternion=[1 0 0 0]
  Selector : Selector  InputPortWidth=6  IndexOptions=Index vector (dialog)  Indices=[1:3]  OutputSizes=1
  Selector1 : Selector  InputPortWidth=6  IndexOptions=Index vector (dialog)  Indices=[4:6]  OutputSizes=1
  Simulink-PS Converter1 : nesl_utility/Simulink-PS Converter  PhysicalDomain=network_engine_domain  SubClassName=ps_input  LeftPortType=input  RightPortType=output  PseudoPeriodic=off  Frequencies=[]  NoiseDistribution=none  NoiseParameters=[]  Unit=1  AffineConversion=off  FilteringAndDerivatives=zero  SimscapeFilterOrder=1  InputFilterTimeConstant=0.001  UdotUserProvided=1
  Simulink-PS Converter2 : nesl_utility/Simulink-PS Converter  PhysicalDomain=network_engine_domain  SubClassName=ps_input  LeftPortType=input  RightPortType=output  PseudoPeriodic=off  Frequencies=[]  NoiseDistribution=none  NoiseParameters=[]  Unit=1  AffineConversion=off  FilteringAndDerivatives=zero  SimscapeFilterOrder=1  InputFilterTimeConstant=0.001  UdotUserProvided=1
  World Frame : sm_lib/Frames and Transforms/World Frame
  Conn Free Surface : PMIOPort  Side=Right
  Response : Outport
  wires:
  Total Force/1 -> Selector1/1, Selector/1
  Selector/1 -> Simulink-PS Converter1/1
  Selector1/1 -> Simulink-PS Converter2/1
  Motion Sensor/1 -> Response/1
  connections:
  External Force and Torque/LConn1 -- Simulink-PS Converter1/RConn1
  External Force and Torque/LConn2 -- Simulink-PS Converter2/RConn1
  Rigid Transform (Setup Initial Disp)/RConn1 -- Body Properties/RConn1 -- Motion Sensor/RConn1 -- External Force and Torque/RConn1
  Conn Free Surface/RConn1 -- Rigid Transform (Setup CG)/LConn1
  Rigid Transform (Setup Initial Disp)/LConn1 -- Rigid Transform (Setup CG)/RConn1
  Motion Sensor/LConn1 -- World Frame/RConn1

== system oc4_VarMass/Float/Hydrodynamic Body/Additional Linear Damping Force Calculation ==
  note: F_damping = c*v
  Velocity : Inport
  linearDamping : Inport  Port=2
  Product1 : Product  Multiplication=Matrix(*)
  F_LinearDamping : Outport
  wires:
  linearDamping/1 -> Product1/1
  Velocity/1 -> Product1/2  "v"
  Product1/1 -> F_LinearDamping/1  "F_LinearDamping"

== system oc4_VarMass/Float/Hydrodynamic Body/B2B Subsystem ==
  note: 1) Add Subsystem or Model blocks as valid variant choices.
      | 2) You cannot connect blocks at this level. At simulation, connectivity is automatically
      | determined, based on the active variant and port name matching.
  note: If simu.b2b == 0, no body to body interaction is used (noB2B)
      | If simu.b2b == 1, use body to body interaction (B2B)
  vel_in : Inport
  acc_in : Inport  Port=2
  B2B : Subsystem  VariantControl=sv_B2B
  noB2B : Subsystem  VariantControl=sv_noB2B
  vel : Outport
  acc : Outport  Port=2

== system oc4_VarMass/Float/Hydrodynamic Body/Hydrostatic Restoring Force Calculation ==
  Displacement : Inport
  Wave Elv : Inport  Port=2
  Add : Sum  Inputs=+-
  Bus Selector : BusSelector  OutputSignals=centerGravity
  Constant : Constant  Value=zeros(1,body.dof-3)
  Linear and Nonlinear Restoring Force Variant Subsystem : Subsystem  Variant=on
  Mux : Mux  Inputs=2
  F_Restoring : Outport
  wires:
  [body1_hydroForce] -> Bus Selector/1
  Add/1 -> Linear and Nonlinear Restoring Force Variant Subsystem/1(In1)  "x_cg"
  Wave Elv/1 -> Linear and Nonlinear Restoring Force Variant Subsystem/2(In2)
  Constant/1 -> Mux/2
  Bus Selector/1 -> Mux/1  "<centerGravity>"
  Mux/1 -> Add/2
  Linear and Nonlinear Restoring Force Variant Subsystem/1(Out1) -> F_Restoring/1  "F_Restoring"
  Displacement/1 -> Add/1  "x"

== system oc4_VarMass/Float/Hydrodynamic Body/Morison Element and Viscous Damping Force Calculation ==
  note: The output force is a combination of the quadratic viscous drag force and the Morison element force.
      |
      | F_quadraticViscous = 0.5*Cd*rho*A*v*|v|
  Displacement : Inport
  Acceleration : Inport  Port=2
  Velocity : Inport  Port=3
  Time : Inport  Port=4
  quadDrag : Inport  Port=5
  Abs1 : Abs  SaturateOnIntegerOverflow=off
  Morison Element Variant Subsystem : Subsystem  Variant=on
  Product : Product
  Product1 : Product  Multiplication=Matrix(*)
  Transport Delay : TransportDelay  DelayTime=10e-8
  "VisSum " : Sum  Inputs=+-
  F_MorisonAndViscous : Outport
  wires:
  quadDrag/1 -> Product1/1  "quadDrag = 0.5 * cd * rho *A"
  Morison Element Variant Subsystem/1(morison_force) -> "VisSum "/2
  Velocity/1 -> Abs1/1, Morison Element Variant Subsystem/2(velocity), Product/1
  Transport Delay/1 -> Morison Element Variant Subsystem/3(acceleration)
  Displacement/1 -> Morison Element Variant Subsystem/1(displacement)
  Time/1 -> Morison Element Variant Subsystem/4(time)
  Product/1 -> Product1/2  "v * |v|"
  Product1/1 -> "VisSum "/1  "F_quadraticViscous"
  Abs1/1 -> Product/2
  Acceleration/1 -> Transport Delay/1
  "VisSum "/1 -> F_MorisonAndViscous/1  "F_MorisonAndViscous"

== system oc4_VarMass/Float/Hydrodynamic Body/Nonlinear Wave Elevation ==
  Displacement : Inport
  Time : Inport  Port=2
  Add : Sum  Inputs=+-
  Center of Gravity : Constant  Value=body.centerGravity
  Constant : Constant  Value=zeros(1,body.dof-3)
  Linear or Instantaneous Free Surface : Subsystem  Variant=on
  Mux : Mux  Inputs=2
  Wave Elevation : Outport
  wires:
  Time/1 -> Linear or Instantaneous Free Surface/2(In2)
  Constant/1 -> Mux/2
  Center of Gravity/1 -> Mux/1  "cg"
  Mux/1 -> Add/2
  Add/1 -> Linear or Instantaneous Free Surface/1(In1)  "x_cg"
  Linear or Instantaneous Free Surface/1(Out1) -> Wave Elevation/1
  Displacement/1 -> Add/1  "x"

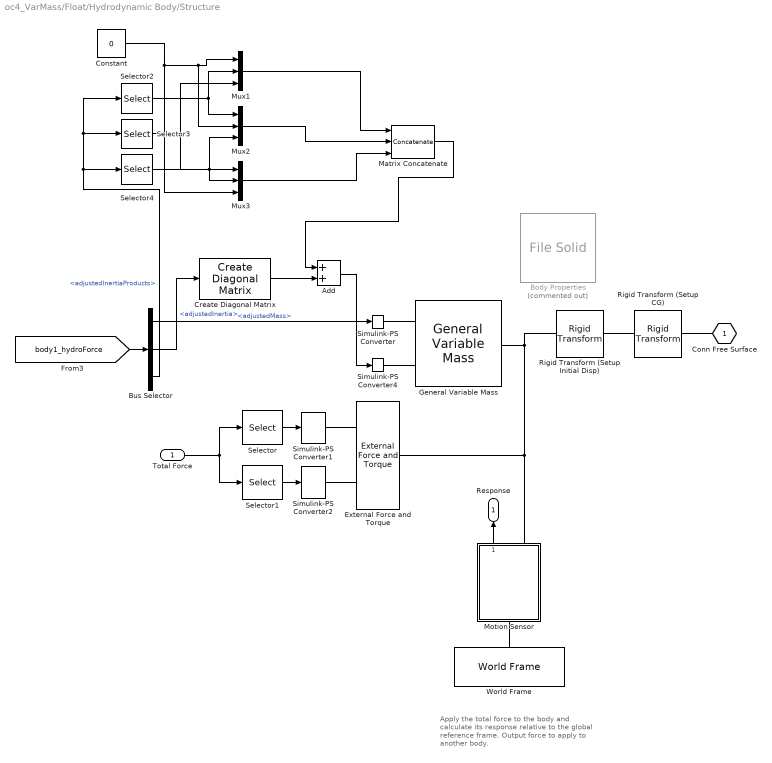
== system oc4_VarMass/Float/Hydrodynamic Body/Structure ==
  note: Apply the total force to the body and calculate its response relative to the global reference frame.
      |
      | Output force to apply to another body.
  Total Force : Inport
  Add : Sum
  Body Properties : sm_lib/Body Elements/File Solid  Commented=on  ExtGeomFileName=../BEM/OC4_Semisub.stl  UnitType=Custom  ExtGeomFileUnits=m  StepReaderType=HEX  ExportConvexHullGeometry=off  InertiaType=Custom  BasedOnType=Density  Density=1000  DensityUnits=kg/(m^3)  Mass=body.hydroForce.(['hf' num2str(body.variableHydro.hydroForceIndexInitial)]).adjustedMass  MassUnits=kg  CenterOfMass=[0 0 0]  CenterOfMassUnits=m  MomentsOfInertia=body.hydroForce.(['hf' num2str(body.variableHydro.hydroForceIndexInitial)]).adjustedInertia  MomentsOfInertiaUnits=kg*m^2  ProductsOfInertia=body.hydroForce.(['hf' num2str(body.variableHydro.hydroForceIndexInitial)]).adjustedInertiaProducts  ProductsOfInertiaUnits=kg*m^2  GraphicType=FromGeometry  MarkerShape=Sphere  MarkerSize=10  GraphicVisPropType=SimpleVisualProperties  GraphicDiffuseColor=body.viz.color  GraphicOpacity=body.viz.opacity  GraphicSpecularColor=[0.5 0.5 0.5 1.0]  GraphicAmbientColor=[0.15 0.15 0.15 1.0]  GraphicEmissiveColor=[0.0 0.0 0.0 1.0]  GraphicShininess=75  DoExposeReferenceFrame=on  SerializedFrames=<Frames/>
  Bus Selector : BusSelector  OutputSignals=adjustedMass,adjustedInertia,adjustedInertiaProducts
  Constant : Constant  Value=0
  Create Diagonal Matrix : matrix_library/Create Diagonal Matrix
      settings: LibrarySourceBlock=|
      | simulink/Matrix
      | Operations/Create Diagonal
      | Matrix
  External Force and Torque : sm_lib/Forces and Torques/External Force and Torque  EnableForceX=off  EnableForceY=off  EnableForceZ=off  EnableForce=on  ForceResolutionFrame=World  EnableTorqueX=off  EnableTorqueY=off  EnableTorqueZ=off  EnableTorque=on  TorqueResolutionFrame=World
  General Variable Mass : sm_lib/Body Elements/Variable Mass/General Variable Mass  VariableInertiaType=Custom  MassType=TimeVarying  Mass=1  MassUnits=kg  CenterOfMassType=Constant  CenterOfMass=[0 0 0]  CenterOfMassUnits=m  InertiaMatrixType=TimeVarying  MomentsOfInertia=[1 1 1]  MomentsOfInertiaUnits=kg*m^2  ProductsOfInertia=[0 0 0]  ProductsOfInertiaUnits=kg*m^2  GraphicType=InertiaEllipsoid  MarkerShape=Sphere  MarkerSize=10  GraphicVisPropType=SimpleVisualProperties  GraphicDiffuseColor=[0.5 0.5 0.5]  GraphicOpacity=1.0  GraphicSpecularColor=[0.5 0.5 0.5 1.0]  GraphicAmbientColor=[0.15 0.15 0.15 1.0]  GraphicEmissiveColor=[0.0 0.0 0.0 1.0]  GraphicShininess=75
  Matrix Concatenate : Concatenate  NumInputs=3  Mode=Multidimensional array  ConcatenateDimension=2
  Motion Sensor : Subsystem
  Mux1 : Mux  Inputs=3
  Mux2 : Mux  Inputs=3
  Mux3 : Mux  Inputs=3
  Rigid Transform (Setup CG) : sm_lib/Frames and Transforms/Rigid Transform  RotationMethod=None  FollAlignAxisA=+X  BaseAlignAxisA=+Y  FollAlignAxisB=+Y  BaseAlignAxisB=+Z  RotationStandardAxis=+Y  RotationAngle=0.05  RotationAngleUnits=rad  RotationArbitraryAxis=[0.57735026918962584 0.57735026918962584 0.57735026918962584]  RotationSequenceAxes=FollowerAxes  RotationSequence=XYX  RotationSequenceAngles=[0 0 0]  RotationSequenceAnglesUnits=deg  RotationMatrix=[1 0 0; 0 1 0; 0 0 1]  Quaternion=[1 0 0 0]  TranslationMethod=Cartesian  TranslationCartesianOffset=body.centerGravity  TranslationCartesianOffsetUnits=m  TranslationStandardAxis=+Z  TranslationStandardOffset=0  TranslationStandardOffsetUnits=m  TranslationROffset=0  TranslationROffsetUnits=m  TranslationThetaOffset=0  TranslationThetaOffsetUnits=deg  TranslationZOffset=0  TranslationZOffsetUnits=m
  Rigid Transform (Setup Initial Disp) : sm_lib/Frames and Transforms/Rigid Transform  RotationMethod=ArbitraryAxis  FollAlignAxisA=+X  BaseAlignAxisA=+Y  FollAlignAxisB=+Y  BaseAlignAxisB=+Z  RotationStandardAxis=+Y  RotationAngle=body.initial.angle  RotationAngleUnits=rad  RotationArbitraryAxis=body.initial.axis  RotationSequenceAxes=FollowerAxes  RotationSequence=XYX  RotationSequenceAngles=[0 0 0]  RotationSequenceAnglesUnits=deg  RotationMatrix=[1 0 0; 0 1 0; 0 0 1]  Quaternion=[1 0 0 0]  TranslationMethod=Cartesian  TranslationCartesianOffset=body.initial.displacement  TranslationCartesianOffsetUnits=m  TranslationStandardAxis=+Z  TranslationStandardOffset=0  TranslationStandardOffsetUnits=m  TranslationROffset=0  TranslationROffsetUnits=m  TranslationThetaOffset=0  TranslationThetaOffsetUnits=deg  TranslationZOffset=0  TranslationZOffsetUnits=m
  Selector : Selector  InputPortWidth=6  IndexOptions=Index vector (dialog)  Indices=[1:3]  OutputSizes=1
  Selector1 : Selector  InputPortWidth=6  IndexOptions=Index vector (dialog)  Indices=[4:6]  OutputSizes=1
  Selector2 : Selector  InputPortWidth=3  IndexOptions=Index vector (dialog)  Indices=1  OutputSizes=1
  Selector3 : Selector  InputPortWidth=3  IndexOptions=Index vector (dialog)  Indices=2  OutputSizes=1
  Selector4 : Selector  InputPortWidth=3  IndexOptions=Index vector (dialog)  Indices=3  OutputSizes=1
  Simulink-PS Converter : nesl_utility/Simulink-PS Converter  PhysicalDomain=network_engine_domain  SubClassName=ps_input  LeftPortType=input  RightPortType=output  PseudoPeriodic=off  Frequencies=[]  NoiseDistribution=none  NoiseParameters=[]  Unit=1  AffineConversion=off  FilteringAndDerivatives=provide  SimscapeFilterOrder=1  InputFilterTimeConstant=0.001  UdotUserProvided=0
  Simulink-PS Converter1 : nesl_utility/Simulink-PS Converter  PhysicalDomain=network_engine_domain  SubClassName=ps_input  LeftPortType=input  RightPortType=output  PseudoPeriodic=off  Frequencies=[]  NoiseDistribution=none  NoiseParameters=[]  Unit=1  AffineConversion=off  FilteringAndDerivatives=zero  SimscapeFilterOrder=1  InputFilterTimeConstant=0.001  UdotUserProvided=1
  Simulink-PS Converter2 : nesl_utility/Simulink-PS Converter  PhysicalDomain=network_engine_domain  SubClassName=ps_input  LeftPortType=input  RightPortType=output  PseudoPeriodic=off  Frequencies=[]  NoiseDistribution=none  NoiseParameters=[]  Unit=1  AffineConversion=off  FilteringAndDerivatives=zero  SimscapeFilterOrder=1  InputFilterTimeConstant=0.001  UdotUserProvided=1
  Simulink-PS Converter4 : nesl_utility/Simulink-PS Converter  PhysicalDomain=network_engine_domain  SubClassName=ps_input  LeftPortType=input  RightPortType=output  PseudoPeriodic=off  Frequencies=[]  NoiseDistribution=none  NoiseParameters=[]  Unit=1  AffineConversion=off  FilteringAndDerivatives=provide  SimscapeFilterOrder=1  InputFilterTimeConstant=0.001  UdotUserProvided=0
  World Frame : sm_lib/Frames and Transforms/World Frame
  Conn Free Surface : PMIOPort  Side=Right
  Response : Outport
  wires:
  Total Force/1 -> Selector1/1, Selector/1
  Selector/1 -> Simulink-PS Converter1/1
  Selector1/1 -> Simulink-PS Converter2/1
  Motion Sensor/1(Response) -> Response/1
  Bus Selector/3 -> Selector4/1, Selector3/1, Selector2/1  "<adjustedInertiaProducts>"
  Selector4/1 -> Mux3/2, Mux2/3
  [body1_hydroForce] -> Bus Selector/1
  Add/1 -> Simulink-PS Converter4/1
  Selector3/1 -> Mux3/1, Mux1/3
  Bus Selector/1 -> Simulink-PS Converter/1  "<adjustedMass>"
  Mux2/1 -> Matrix Concatenate/2
  Mux3/1 -> Matrix Concatenate/3
  Mux1/1 -> Matrix Concatenate/1
  Matrix Concatenate/1 -> Add/1
  Constant/1 -> Mux3/3, Mux1/1, Mux2/2
  Selector2/1 -> Mux2/1, Mux1/2
  Create Diagonal Matrix/1 -> Add/2
  Bus Selector/2 -> Create Diagonal Matrix/1  "<adjustedInertia>"
  connections:
  External Force and Torque/LConn1 -- Simulink-PS Converter1/RConn1
  External Force and Torque/LConn2 -- Simulink-PS Converter2/RConn1
  Rigid Transform (Setup Initial Disp)/RConn1 -- General Variable Mass/RConn1 -- External Force and Torque/RConn1 -- Motion Sensor/RConn1
  Conn Free Surface/RConn1 -- Rigid Transform (Setup CG)/LConn1
  Rigid Transform (Setup Initial Disp)/LConn1 -- Rigid Transform (Setup CG)/RConn1
  World Frame/RConn1 -- Motion Sensor/LConn1
  Simulink-PS Converter/RConn1 -- General Variable Mass/LConn1
  Simulink-PS Converter4/RConn1 -- General Variable Mass/LConn2
